simulink model "tip_assist_lib_bucket_target_compensation"  (Simulink 9.0)
settings: Solver=VariableStepAuto  StartTime=0.0  StopTime=10.0  RelTol=1e-3
settings Model: Creator=CurriSD  LastModifiedBy=CurriSD
settings DataIOCC: SaveFormat=Dataset
settings OptimizationCC: LifeSpan=auto
settings DebuggingCC: UnderspecifiedInitializationDetection=Simplified  MergeDetectMultiDrivingBlocksExec=error  SFUnexpectedBacktrackingDiag=error  SFNoUnconditionalDefaultTransitionDiag=error  SFExecutionAtInitializationDiag=warning
settings HardwareCC: ProdBitPerPointer=64  ProdBitPerSizeT=64  ProdBitPerPtrDiffT=64  ProdLargestAtomicFloat=Float  ProdIntDivRoundTo=Zero  ProdEndianess=LittleEndian  ProdWordSize=64  ProdHWDeviceType=Intel->x86-64 (Windows64)
settings ModelReferenceCC: PropagateSignalLabelsOutOfModel=on
settings CodeAppCC: StateflowObjectComments=off
settings GRTTargetCC: TargetLangStandard=C99 (ISO)
settings ConfigComp: CovMetricSettings=dwe  CovHtmlReporting=off  CovSaveCumulativeToWorkspaceVar=off  CovSaveSingleToWorkspaceVar=off  CovExternalEMLEnable=on

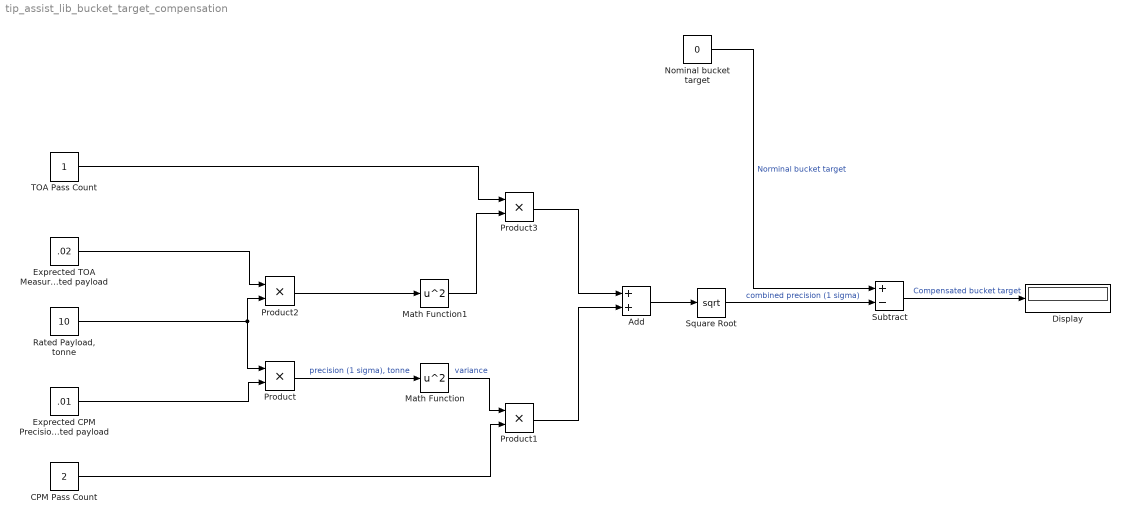
== system tip_assist_lib_bucket_target_compensation ==
  Add : Sum
  CPM Pass Count : Constant  Value=2
  Display : Display
  "Exprected CPM Precision (1 sigma), pct of rated payload" : Constant  Value=.01
  "Exprected TOA Measurement Precision (1 sigma), pct of rated payload" : Constant  Value=.02
  Math Function : Math  Operator=square  SaturateOnIntegerOverflow=on
  Math Function1 : Math  Operator=square  SaturateOnIntegerOverflow=on
  Nominal bucket target : Constant  Value=0
  Product{,1..3} (4 alike) : Product
  "Rated Payload, tonne" : Constant  Value=10
  Square Root : Sqrt  SaturateOnIntegerOverflow=on
  Subtract : Sum  Inputs=+-
  TOA Pass Count : Constant
  wires:
  "Exprected CPM Precision (1 sigma), pct of rated payload"/1 -> Product/2
  "Rated Payload, tonne"/1 -> Product2/2, Product/1
  Product/1 -> Math Function/1  "precision (1 sigma), tonne"
  CPM Pass Count/1 -> Product1/2
  Math Function/1 -> Product1/1  "variance"
  Product1/1 -> Add/2
  "Exprected TOA Measurement Precision (1 sigma), pct of rated payload"/1 -> Product2/1
  Product2/1 -> Math Function1/1
  Math Function1/1 -> Product3/2
  TOA Pass Count/1 -> Product3/1
  Product3/1 -> Add/1
  Add/1 -> Square Root/1
  Square Root/1 -> Subtract/2  "combined precision (1 sigma)"
  Nominal bucket target/1 -> Subtract/1  "Norminal bucket target"
  Subtract/1 -> Display/1  "Compensated bucket target"
